simulink model "PX4_Receive"  (R2025b)
settings: Solver=FixedStepAuto  StartTime=0.0  StopTime=60  RelTol=1e-3
undefined symbols (not defined in the file or in its folder): acceleration, actuator, attitude, body_rate, codertarget, command, control, CustomLQR, FlightPlan, from_external, gcbh, HomeNED, HoverThrust, jerk, param1, param2, param3, pitch, pitch_body, position, PX4Params, PX4Tune, q_d, roll, roll_body, source_component, source_system, target_component, target_system, TestAmplitude, TestAxis, thrust_body, timestamp, timestamp_sample, TUNING_ON, TuningMaxClimbRate, TuningMinAltitude, TuningStage, TuningTestStart, velocity, yaw, yaw_body, yaw_sp_move_rate, yawspeed
libraries: px4Utilslib x53, px4uORBlib x52, simulink x13
(part 2 of 2)

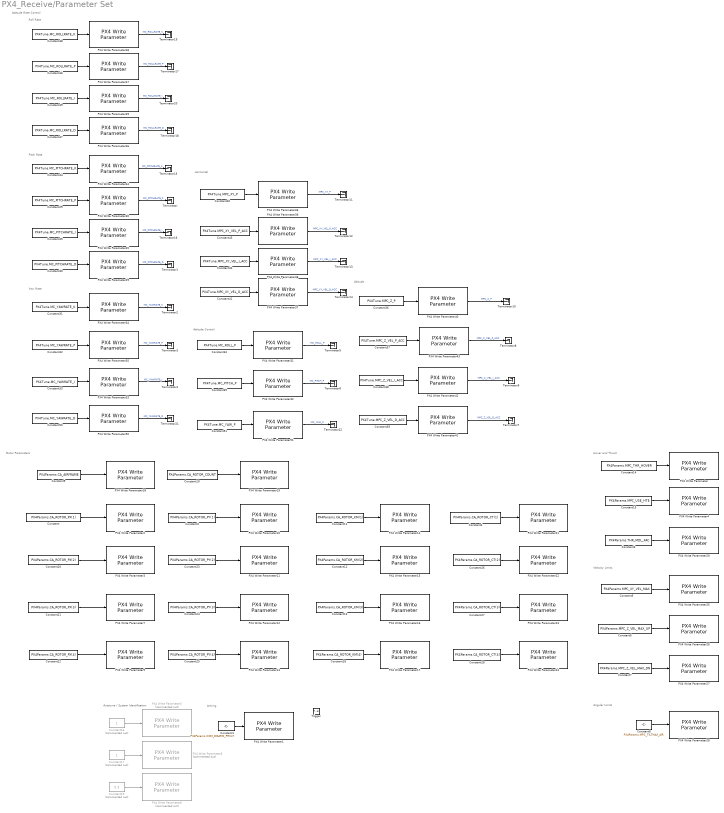
== system PX4_Receive/Parameter Set ==
  note: Yaw Rate
  note: Roll Rate
  note: Pitch Rate
  note: Horizontal
  note: Altitude
  note: Attitude Rate Control
  note: Arming
  note: Autotune / System Identification
  note: Hover and Thrust
  note: Motor Parameters
  note: Velocity Limits
  note: Angular Limits
  note: Attitude Control
  Trigger : TriggerPort  VariantControl=(inherit)  ShowOutputPort=on  PortDimensions=1
  Constant : Constant  Value=PX4Params.CA_ROTOR_PX(1)  OutDataTypeStr=single
  Constant1 : Constant  Value=PX4Params.COM_DISARM_PRFLT  OutDataTypeStr=single
  Constant10 : Constant  Value=PX4Params.CA_ROTOR_COUNT  OutDataTypeStr=int32
  Constant11 : Constant  Value=PX4Params.CA_ROTOR_KM(1)  OutDataTypeStr=single
  Constant12 : Constant  Value=PX4Params.CA_ROTOR_KM(2)  OutDataTypeStr=single
  Constant13 : Constant  Value=PX4Params.CA_ROTOR_KM(3)  OutDataTypeStr=single
  Constant14 : Constant  Value=PX4Params.MPC_THR_HOVER  OutDataTypeStr=single
  Constant15 : Constant  Value=PX4Params.MPC_USE_HTE  OutDataTypeStr=int32
  Constant16 : Constant  Commented=on  OutDataTypeStr=int32
  Constant17 : Constant  Commented=on  OutDataTypeStr=int32
  Constant18 : Constant  Value=PX4Params.CA_ROTOR_KM(4)  OutDataTypeStr=single
  Constant19 : Constant  Commented=on  Value=0.3  OutDataTypeStr=single
  Constant2 : Constant  Value=PX4Params.CA_ROTOR_PY(1)  OutDataTypeStr=single
  Constant20 : Constant  Value=PX4Params.CA_ROTOR_PX(2)  OutDataTypeStr=single
  Constant21 : Constant  Value=PX4Params.CA_ROTOR_PX(3)  OutDataTypeStr=single
  Constant22 : Constant  Value=PX4Params.CA_ROTOR_PX(4)  OutDataTypeStr=single
  Constant23 : Constant  Value=PX4Params.CA_ROTOR_PY(2)  OutDataTypeStr=single
  Constant24 : Constant  Value=PX4Params.CA_ROTOR_PY(3)  OutDataTypeStr=single
  Constant25 : Constant  Value=PX4Params.CA_ROTOR_PY(4)  OutDataTypeStr=single
  Constant26 : Constant  Value=PX4Params.CA_ROTOR_CT(2)  OutDataTypeStr=single
  Constant27 : Constant  Value=PX4Params.CA_ROTOR_CT(3)  OutDataTypeStr=single
  Constant28 : Constant  Value=PX4Params.CA_ROTOR_CT(4)  OutDataTypeStr=single
  Constant29 : Constant  Value=PX4Tune.MC_PITCHRATE_P  OutDataTypeStr=single
  Constant3 : Constant  Value=PX4Params.THR_MDL_FAC  OutDataTypeStr=single
  Constant30 : Constant  Value=PX4Tune.MC_PITCHRATE_D  OutDataTypeStr=single
  Constant31 : Constant  Value=PX4Tune.MC_YAWRATE_K  OutDataTypeStr=single
  Constant32 : Constant  Value=PX4Tune.MC_YAWRATE_P  OutDataTypeStr=single
  Constant33 : Constant  Value=PX4Tune.MC_YAWRATE_I  OutDataTypeStr=single
  Constant34 : Constant  Value=PX4Tune.MC_ROLL_P  OutDataTypeStr=single
  Constant35 : Constant  Value=PX4Tune.MC_PITCH_P  OutDataTypeStr=single
  Constant36 : Constant  Value=PX4Tune.MPC_Z_P  OutDataTypeStr=single
  Constant37 : Constant  Value=PX4Tune.MPC_Z_VEL_P_ACC  OutDataTypeStr=single
  Constant38 : Constant  Value=PX4Tune.MPC_Z_VEL_I_ACC  OutDataTypeStr=single
  Constant39 : Constant  Value=PX4Tune.MPC_Z_VEL_D_ACC  OutDataTypeStr=single
  Constant4 : Constant  Value=PX4Params.CA_ROTOR_CT(1)  OutDataTypeStr=single
  Constant40 : Constant  Value=PX4Tune.MPC_XY_P  OutDataTypeStr=single
  Constant41 : Constant  Value=PX4Tune.MPC_XY_VEL_D_ACC  OutDataTypeStr=single
  Constant42 : Constant  Value=PX4Tune.MPC_XY_VEL_I_ACC  OutDataTypeStr=single
  Constant43 : Constant  Value=PX4Tune.MPC_XY_VEL_P_ACC  OutDataTypeStr=single
  Constant44 : Constant  Value=PX4Tune.MC_PITCHRATE_K  OutDataTypeStr=single
  Constant45 : Constant  Value=PX4Tune.MC_PITCHRATE_I  OutDataTypeStr=single
  Constant46 : Constant  Value=PX4Tune.MC_ROLLRATE_P  OutDataTypeStr=single
  Constant47 : Constant  Value=PX4Tune.MC_ROLLRATE_D  OutDataTypeStr=single
  Constant48 : Constant  Value=PX4Tune.MC_ROLLRATE_K  OutDataTypeStr=single
  Constant49 : Constant  Value=PX4Tune.MC_ROLLRATE_I  OutDataTypeStr=single
  Constant5 : Constant  Value=PX4Params.MPC_XY_VEL_MAX  OutDataTypeStr=single
  Constant50 : Constant  Value=PX4Tune.MC_YAWRATE_D  OutDataTypeStr=single
  Constant51 : Constant  Value=PX4Tune.MC_YAW_P  OutDataTypeStr=single
  Constant6 : Constant  Value=PX4Params.MPC_Z_VEL_MAX_UP  OutDataTypeStr=single
  Constant7 : Constant  Value=PX4Params.MPC_Z_VEL_MAX_DN  OutDataTypeStr=single
  Constant8 : Constant  Value=PX4Params.MPC_TILTMAX_AIR  OutDataTypeStr=single
  Constant9 : Constant  Value=PX4Params.CA_AIRFRAME  OutDataTypeStr=int32
  PX4 Write Parameter : px4Utilslib/PX4 Write Parameter  ParameterName=MPC_THR_HOVER  outputStatus=off  SimulateUsing=Code generation
  PX4 Write Parameter1 : px4Utilslib/PX4 Write Parameter  ParameterName=COM_DISARM_PRFLT  outputStatus=off  SimulateUsing=Code generation
  PX4 Write Parameter10 : px4Utilslib/PX4 Write Parameter  ParameterName=CA_ROTOR0_PY  outputStatus=off  SimulateUsing=Code generation
  PX4 Write Parameter11 : px4Utilslib/PX4 Write Parameter  ParameterName=CA_ROTOR1_PY  outputStatus=off  SimulateUsing=Code generation
  PX4 Write Parameter12 : px4Utilslib/PX4 Write Parameter  ParameterName=CA_ROTOR2_PY  outputStatus=off  SimulateUsing=Code generation
  PX4 Write Parameter13 : px4Utilslib/PX4 Write Parameter  ParameterName=CA_ROTOR3_PY  outputStatus=off  SimulateUsing=Code generation
  PX4 Write Parameter14 : px4Utilslib/PX4 Write Parameter  ParameterName=CA_ROTOR0_KM  outputStatus=off  SimulateUsing=Code generation
  PX4 Write Parameter15 : px4Utilslib/PX4 Write Parameter  ParameterName=CA_ROTOR1_KM  outputStatus=off  SimulateUsing=Code generation
  PX4 Write Parameter16 : px4Utilslib/PX4 Write Parameter  ParameterName=CA_ROTOR2_KM  outputStatus=off  SimulateUsing=Code generation
  PX4 Write Parameter17 : px4Utilslib/PX4 Write Parameter  ParameterName=CA_ROTOR3_KM  outputStatus=off  SimulateUsing=Code generation
  PX4 Write Parameter18 : px4Utilslib/PX4 Write Parameter  ParameterName=CA_AIRFRAME  outputStatus=off  SimulateUsing=Code generation
  PX4 Write Parameter19 : px4Utilslib/PX4 Write Parameter  ParameterName=CA_ROTOR_COUNT  outputStatus=off  SimulateUsing=Code generation
  PX4 Write Parameter2 : px4Utilslib/PX4 Write Parameter  ParameterName=CA_ROTOR0_PX  outputStatus=off  SimulateUsing=Code generation
  PX4 Write Parameter20 : px4Utilslib/PX4 Write Parameter  ParameterName=THR_MDL_FAC  outputStatus=off  SimulateUsing=Code generation
  PX4 Write Parameter21 : px4Utilslib/PX4 Write Parameter  ParameterName=CA_ROTOR0_CT  outputStatus=off  SimulateUsing=Code generation
  PX4 Write Parameter22 : px4Utilslib/PX4 Write Parameter  ParameterName=CA_ROTOR1_CT  outputStatus=off  SimulateUsing=Code generation
  PX4 Write Parameter23 : px4Utilslib/PX4 Write Parameter  ParameterName=CA_ROTOR2_CT  outputStatus=off  SimulateUsing=Code generation
  PX4 Write Parameter24 : px4Utilslib/PX4 Write Parameter  ParameterName=CA_ROTOR3_CT  outputStatus=off  SimulateUsing=Code generation
  PX4 Write Parameter25 : px4Utilslib/PX4 Write Parameter  ParameterName=MPC_XY_VEL_MAX  outputStatus=off  SimulateUsing=Code generation
  PX4 Write Parameter26 : px4Utilslib/PX4 Write Parameter  ParameterName=MPC_Z_VEL_MAX_UP  outputStatus=off  SimulateUsing=Code generation
  PX4 Write Parameter27 : px4Utilslib/PX4 Write Parameter  ParameterName=MPC_Z_VEL_MAX_DN  outputStatus=off  SimulateUsing=Code generation
  PX4 Write Parameter28 : px4Utilslib/PX4 Write Parameter  ParameterName=MPC_TILTMAX_AIR  outputStatus=off  SimulateUsing=Code generation
  PX4 Write Parameter29 : px4Utilslib/PX4 Write Parameter  ParameterName=MC_PITCHRATE_D  outputStatus=on  SimulateUsing=Code generation
  PX4 Write Parameter3 : px4Utilslib/PX4 Write Parameter  ParameterName=CA_ROTOR1_PX  outputStatus=off  SimulateUsing=Code generation
  PX4 Write Parameter30 : px4Utilslib/PX4 Write Parameter  ParameterName=MC_PITCHRATE_P  outputStatus=on  SimulateUsing=Code generation
  PX4 Write Parameter31 : px4Utilslib/PX4 Write Parameter  ParameterName=MC_ROLL_P  outputStatus=on  SimulateUsing=Code generation
  PX4 Write Parameter32 : px4Utilslib/PX4 Write Parameter  ParameterName=MC_PITCH_P  outputStatus=on  SimulateUsing=Code generation
  PX4 Write Parameter33 : px4Utilslib/PX4 Write Parameter  ParameterName=MC_YAWRATE_I  outputStatus=on  SimulateUsing=Code generation
  PX4 Write Parameter34 : px4Utilslib/PX4 Write Parameter  ParameterName=MC_YAWRATE_K  outputStatus=on  SimulateUsing=Code generation
  PX4 Write Parameter35 : px4Utilslib/PX4 Write Parameter  ParameterName=MC_YAWRATE_P  outputStatus=on  SimulateUsing=Code generation
  PX4 Write Parameter36 : px4Utilslib/PX4 Write Parameter  ParameterName=MPC_XY_P  outputStatus=on  SimulateUsing=Code generation
  PX4 Write Parameter37 : px4Utilslib/PX4 Write Parameter  ParameterName=MPC_XY_VEL_D_ACC  outputStatus=on  SimulateUsing=Code generation
  PX4 Write Parameter38 : px4Utilslib/PX4 Write Parameter  ParameterName=MPC_XY_VEL_I_ACC  outputStatus=on  SimulateUsing=Code generation
  PX4 Write Parameter39 : px4Utilslib/PX4 Write Parameter  ParameterName=MPC_XY_VEL_P_ACC  outputStatus=on  SimulateUsing=Code generation
  PX4 Write Parameter4 : px4Utilslib/PX4 Write Parameter  ParameterName=MPC_USE_HTE  outputStatus=off  SimulateUsing=Code generation
  PX4 Write Parameter40 : px4Utilslib/PX4 Write Parameter  ParameterName=MPC_Z_P  outputStatus=on  SimulateUsing=Code generation
  PX4 Write Parameter41 : px4Utilslib/PX4 Write Parameter  ParameterName=MPC_Z_VEL_D_ACC  outputStatus=on  SimulateUsing=Code generation
  PX4 Write Parameter42 : px4Utilslib/PX4 Write Parameter  ParameterName=MPC_Z_VEL_I_ACC  outputStatus=on  SimulateUsing=Code generation
  PX4 Write Parameter43 : px4Utilslib/PX4 Write Parameter  ParameterName=MPC_Z_VEL_P_ACC  outputStatus=on  SimulateUsing=Code generation
  PX4 Write Parameter44 : px4Utilslib/PX4 Write Parameter  ParameterName=MC_PITCHRATE_K  outputStatus=on  SimulateUsing=Code generation
  PX4 Write Parameter45 : px4Utilslib/PX4 Write Parameter  ParameterName=MC_PITCHRATE_I  outputStatus=on  SimulateUsing=Code generation
  PX4 Write Parameter46 : px4Utilslib/PX4 Write Parameter  ParameterName=MC_ROLLRATE_D  outputStatus=on  SimulateUsing=Code generation
  PX4 Write Parameter47 : px4Utilslib/PX4 Write Parameter  ParameterName=MC_ROLLRATE_P  outputStatus=on  SimulateUsing=Code generation
  PX4 Write Parameter48 : px4Utilslib/PX4 Write Parameter  ParameterName=MC_ROLLRATE_K  outputStatus=on  SimulateUsing=Code generation
  PX4 Write Parameter49 : px4Utilslib/PX4 Write Parameter  ParameterName=MC_ROLLRATE_I  outputStatus=on  SimulateUsing=Code generation
  PX4 Write Parameter5 : px4Utilslib/PX4 Write Parameter  Commented=on  ParameterName=MC_AT_EN  outputStatus=off  SimulateUsing=Code generation
  PX4 Write Parameter50 : px4Utilslib/PX4 Write Parameter  ParameterName=MC_YAWRATE_D  outputStatus=on  SimulateUsing=Code generation
  PX4 Write Parameter51 : px4Utilslib/PX4 Write Parameter  ParameterName=MC_YAW_P  outputStatus=on  SimulateUsing=Code generation
  PX4 Write Parameter6 : px4Utilslib/PX4 Write Parameter  Commented=on  ParameterName=MC_AT_APPLY  outputStatus=off  SimulateUsing=Code generation
  PX4 Write Parameter7 : px4Utilslib/PX4 Write Parameter  ParameterName=CA_ROTOR2_PX  outputStatus=off  SimulateUsing=Code generation
  PX4 Write Parameter8 : px4Utilslib/PX4 Write Parameter  Commented=on  ParameterName=MC_AT_SYSID_AMP  outputStatus=off  SimulateUsing=Code generation
  PX4 Write Parameter9 : px4Utilslib/PX4 Write Parameter  ParameterName=CA_ROTOR3_PX  outputStatus=off  SimulateUsing=Code generation
  Terminator{,1..22} (23 alike) : Terminator
  wires:
  Constant19/1 -> PX4 Write Parameter8/1
  Constant17/1 -> PX4 Write Parameter6/1
  Constant14/1 -> PX4 Write Parameter/1
  Constant16/1 -> PX4 Write Parameter5/1
  Constant15/1 -> PX4 Write Parameter4/1
  Constant1/1 -> PX4 Write Parameter1/1
  Constant/1 -> PX4 Write Parameter2/1
  Constant21/1 -> PX4 Write Parameter7/1
  Constant2/1 -> PX4 Write Parameter10/1
  Constant22/1 -> PX4 Write Parameter9/1
  Constant9/1 -> PX4 Write Parameter18/1
  Constant11/1 -> PX4 Write Parameter14/1
  Constant12/1 -> PX4 Write Parameter15/1
  Constant13/1 -> PX4 Write Parameter16/1
  Constant18/1 -> PX4 Write Parameter17/1
  Constant10/1 -> PX4 Write Parameter19/1
  Constant3/1 -> PX4 Write Parameter20/1
  Constant5/1 -> PX4 Write Parameter25/1
  Constant6/1 -> PX4 Write Parameter26/1
  Constant7/1 -> PX4 Write Parameter27/1
  Constant8/1 -> PX4 Write Parameter28/1
  Constant20/1 -> PX4 Write Parameter3/1
  Constant23/1 -> PX4 Write Parameter11/1
  Constant24/1 -> PX4 Write Parameter12/1
  Constant25/1 -> PX4 Write Parameter13/1
  Constant4/1 -> PX4 Write Parameter21/1
  Constant26/1 -> PX4 Write Parameter22/1
  Constant27/1 -> PX4 Write Parameter23/1
  Constant28/1 -> PX4 Write Parameter24/1
  Constant29/1 -> PX4 Write Parameter30/1
  Constant30/1 -> PX4 Write Parameter29/1
  Constant31/1 -> PX4 Write Parameter34/1
  Constant32/1 -> PX4 Write Parameter35/1
  Constant33/1 -> PX4 Write Parameter33/1
  Constant35/1 -> PX4 Write Parameter32/1
  Constant34/1 -> PX4 Write Parameter31/1
  Constant36/1 -> PX4 Write Parameter40/1
  Constant39/1 -> PX4 Write Parameter41/1
  Constant38/1 -> PX4 Write Parameter42/1
  Constant37/1 -> PX4 Write Parameter43/1
  Constant40/1 -> PX4 Write Parameter36/1
  Constant41/1 -> PX4 Write Parameter37/1
  Constant42/1 -> PX4 Write Parameter38/1
  Constant43/1 -> PX4 Write Parameter39/1
  PX4 Write Parameter30/1 -> Terminator/1  "MC_PITCHRATE_P"
  PX4 Write Parameter29/1 -> Terminator1/1  "MC_PITCHRATE_D"
  PX4 Write Parameter35/1 -> Terminator3/1  "MC_YAWRATE_P"
  PX4 Write Parameter34/1 -> Terminator2/1  "MC_YAWRATE_K"
  PX4 Write Parameter33/1 -> Terminator4/1  "MC_YAWRATE_I"
  PX4 Write Parameter31/1 -> Terminator5/1  "MC_ROLL_P"
  PX4 Write Parameter32/1 -> Terminator6/1  "MC_PITCH_P"
  PX4 Write Parameter43/1 -> Terminator8/1  "MPC_Z_VEL_P_ACC"
  PX4 Write Parameter40/1 -> Terminator10/1  "MPC_Z_P"
  PX4 Write Parameter42/1 -> Terminator9/1  "MPC_Z_VEL_I_ACC"
  PX4 Write Parameter41/1 -> Terminator7/1  "MPC_Z_VEL_D_ACC"
  PX4 Write Parameter36/1 -> Terminator11/1  "MPC_XY_P"
  PX4 Write Parameter39/1 -> Terminator12/1  "MPC_XY_VEL_P_ACC"
  PX4 Write Parameter38/1 -> Terminator13/1  "MPC_XY_VEL_I_ACC"
  PX4 Write Parameter37/1 -> Terminator14/1  "MPC_XY_VEL_D_ACC"
  PX4 Write Parameter44/1 -> Terminator15/1  "MC_PITCHRATE_K"
  Constant44/1 -> PX4 Write Parameter44/1
  Constant45/1 -> PX4 Write Parameter45/1
  PX4 Write Parameter45/1 -> Terminator16/1  "MC_PITCHRATE_I"
  PX4 Write Parameter49/1 -> Terminator20/1  "MC_ROLLRATE_I"
  Constant48/1 -> PX4 Write Parameter48/1
  PX4 Write Parameter46/1 -> Terminator18/1  "MC_ROLLRATE_D"
  Constant47/1 -> PX4 Write Parameter46/1
  PX4 Write Parameter47/1 -> Terminator17/1  "MC_ROLLRATE_P"
  PX4 Write Parameter48/1 -> Terminator19/1  "MC_ROLLRATE_K"
  Constant46/1 -> PX4 Write Parameter47/1
  Constant49/1 -> PX4 Write Parameter49/1
  Constant50/1 -> PX4 Write Parameter50/1
  PX4 Write Parameter50/1 -> Terminator21/1  "MC_YAWRATE_D"
  Constant51/1 -> PX4 Write Parameter51/1
  PX4 Write Parameter51/1 -> Terminator22/1  "MC_YAW_P"

== system PX4_Receive/Custom Controller (LQR)/Disable land auto-disarm ==
  Trigger : TriggerPort  VariantControl=(inherit)  PortDimensions=1
  COM_DISARM_LAND : px4Utilslib/PX4 Write Parameter  ParameterName=COM_DISARM_LAND  outputStatus=off  SimulateUsing=Code generation
  Value : Constant  Value=single(-1)  OutDataTypeStr=single
  wires:
  Value/1 -> COM_DISARM_LAND/1

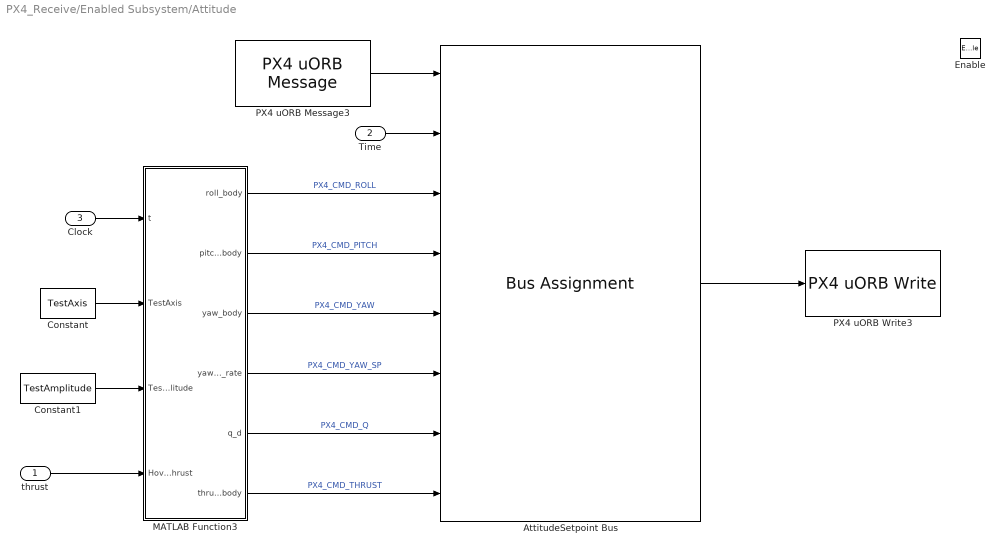
== system PX4_Receive/Enabled Subsystem/Attitude ==
  thrust : Inport
  Time : Inport  Port=2
  Clock : Inport  Port=3
  Enable : EnablePort
  AttitudeSetpoint Bus : BusAssignment  AssignedSignals=timestamp,roll_body,pitch_body,yaw_body,yaw_sp_move_rate,q_d,thrust_body
  Constant : Constant  Value=TestAxis
  Constant1 : Constant  Value=TestAmplitude
  MATLAB Function3 : MATLAB Function  TreatAsAtomicUnit=on
  PX4 uORB Message3 : px4uORBlib/PX4 uORB Message  uORBTopic=VehicleAttitudeSetpoint  SampleTime=-1  selectInstance=vehicle_attitude_setpoint
  PX4 uORB Write3 : px4uORBlib/PX4 uORB Write  uORBTopic=VehicleAttitudeSetpoint  selectInstance=vehicle_attitude_setpoint  MessageQueueLen=1
  wires:
  MATLAB Function3/5(q_d) -> AttitudeSetpoint Bus/7  "PX4_CMD_Q"
  Constant/1 -> MATLAB Function3/2(TestAxis)
  MATLAB Function3/1(roll_body) -> AttitudeSetpoint Bus/3  "PX4_CMD_ROLL"
  PX4 uORB Message3/1 -> AttitudeSetpoint Bus/1
  MATLAB Function3/2(pitch_body) -> AttitudeSetpoint Bus/4  "PX4_CMD_PITCH"
  MATLAB Function3/4(yaw_sp_move_rate) -> AttitudeSetpoint Bus/6  "PX4_CMD_YAW_SP"
  MATLAB Function3/3(yaw_body) -> AttitudeSetpoint Bus/5  "PX4_CMD_YAW"
  Time/1 -> AttitudeSetpoint Bus/2
  AttitudeSetpoint Bus/1 -> PX4 uORB Write3/1
  Constant1/1 -> MATLAB Function3/3(TestAmplitude)
  MATLAB Function3/6(thrust_body) -> AttitudeSetpoint Bus/8  "PX4_CMD_THRUST"
  thrust/1 -> MATLAB Function3/4(HoverThrust)
  Clock/1 -> MATLAB Function3/1(t)

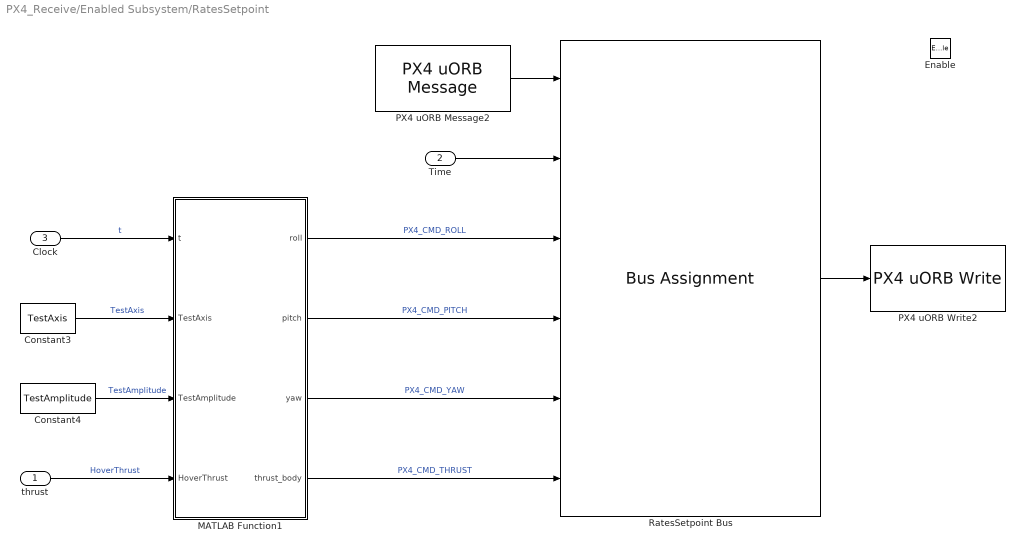
== system PX4_Receive/Enabled Subsystem/RatesSetpoint ==
  thrust : Inport
  Time : Inport  Port=2
  Clock : Inport  Port=3
  Enable : EnablePort
  Constant3 : Constant  Value=TestAxis
  Constant4 : Constant  Value=TestAmplitude
  MATLAB Function1 : MATLAB Function  TreatAsAtomicUnit=on
  PX4 uORB Message2 : px4uORBlib/PX4 uORB Message  uORBTopic=VehicleRatesSetpoint  SampleTime=-1  selectInstance=VehicleRatesSetpoint
  PX4 uORB Write2 : px4uORBlib/PX4 uORB Write  uORBTopic=VehicleRatesSetpoint  selectInstance=VehicleRatesSetpoint  MessageQueueLen=1
  RatesSetpoint Bus : BusAssignment  AssignedSignals=timestamp,roll,pitch,yaw,thrust_body
  wires:
  Time/1 -> RatesSetpoint Bus/2
  thrust/1 -> MATLAB Function1/4(HoverThrust)  "HoverThrust"
  MATLAB Function1/4(thrust_body) -> RatesSetpoint Bus/6  "PX4_CMD_THRUST"
  MATLAB Function1/1(roll) -> RatesSetpoint Bus/3  "PX4_CMD_ROLL"
  Constant4/1 -> MATLAB Function1/3(TestAmplitude)  "TestAmplitude"
  Constant3/1 -> MATLAB Function1/2(TestAxis)  "TestAxis"
  PX4 uORB Message2/1 -> RatesSetpoint Bus/1
  MATLAB Function1/3(yaw) -> RatesSetpoint Bus/5  "PX4_CMD_YAW"
  MATLAB Function1/2(pitch) -> RatesSetpoint Bus/4  "PX4_CMD_PITCH"
  RatesSetpoint Bus/1 -> PX4 uORB Write2/1
  Clock/1 -> MATLAB Function1/1(t)  "t"

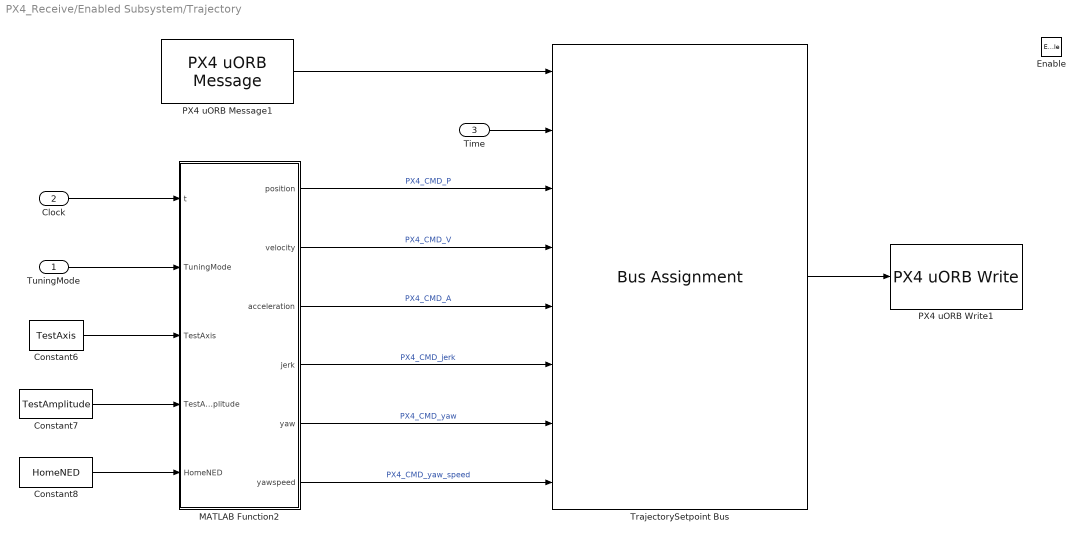
== system PX4_Receive/Enabled Subsystem/Trajectory ==
  TuningMode : Inport
  Clock : Inport  Port=2
  Time : Inport  Port=3
  Enable : EnablePort
  Constant6 : Constant  Value=TestAxis
  Constant7 : Constant  Value=TestAmplitude
  Constant8 : Constant  Value=HomeNED
  MATLAB Function2 : MATLAB Function  TreatAsAtomicUnit=on
  PX4 uORB Message1 : px4uORBlib/PX4 uORB Message  uORBTopic=TrajectorySetpoint  SampleTime=-1  selectInstance=TrajectorySetpoint
  PX4 uORB Write1 : px4uORBlib/PX4 uORB Write  uORBTopic=TrajectorySetpoint  selectInstance=TrajectorySetpoint  MessageQueueLen=1
  TrajectorySetpoint Bus : BusAssignment  AssignedSignals=timestamp,position,velocity,acceleration,jerk,yaw,yawspeed
  wires:
  MATLAB Function2/2(velocity) -> TrajectorySetpoint Bus/4  "PX4_CMD_V"
  Time/1 -> TrajectorySetpoint Bus/2
  Constant8/1 -> MATLAB Function2/5(HomeNED)
  Constant7/1 -> MATLAB Function2/4(TestAmplitude)
  MATLAB Function2/5(yaw) -> TrajectorySetpoint Bus/7  "PX4_CMD_yaw"
  TuningMode/1 -> MATLAB Function2/2(TuningMode)
  MATLAB Function2/6(yawspeed) -> TrajectorySetpoint Bus/8  "PX4_CMD_yaw_speed"
  MATLAB Function2/1(position) -> TrajectorySetpoint Bus/3  "PX4_CMD_P"
  MATLAB Function2/4(jerk) -> TrajectorySetpoint Bus/6  "PX4_CMD_jerk"
  TrajectorySetpoint Bus/1 -> PX4 uORB Write1/1
  PX4 uORB Message1/1 -> TrajectorySetpoint Bus/1
  MATLAB Function2/3(acceleration) -> TrajectorySetpoint Bus/5  "PX4_CMD_A"
  Constant6/1 -> MATLAB Function2/3(TestAxis)
  Clock/1 -> MATLAB Function2/1(t)

== matlab function PX4_Receive/Enabled Subsystem/Attitude/MATLAB Function3 ==
  data: roll_body output; t input; pitch_body output; TestAxis input; TestAmplitude input; HoverThrust input; yaw_body output; yaw_sp_move_rate output; q_d output; thrust_body output

function [roll_body, pitch_body, yaw_body, ...
          yaw_sp_move_rate, q_d, thrust_body] = ...
    attitude_test(t, TestAxis, TestAmplitude, HoverThrust)
%#codegen
% Automated attitude controller tests.
%
% Inputs:
% t             - Elapsed test time [s]
% TestAxis      - 1=Roll, 2=Pitch, 3=Yaw
% TestAmplitude - Attitude amplitude [rad]
% HoverThrust   - Normalized hover thrust magnitude [0,1]

roll_body  = single(0);
pitch_body = single(0);
yaw_body   = single(0);

yaw_sp_move_rate = single(0);

% Positive and negative attitude steps
[axisNow,segmentTime,segmentAmplitude]=px4_tuning_segment(t,uint8(2),TestAxis,TestAmplitude);
cmd=px4_tuning_step_command(segmentTime,uint8(2),segmentAmplitude);

switch axisNow
    case 1
        roll_body = cmd;
    case 2
        pitch_body = cmd;
    case 3
        yaw_body = cmd;
end

% Euler ZYX -> quaternion
% PX4 uses scalar-first ordering [w; x; y; z]

cr = cos(double(roll_body)/2);
sr = sin(double(roll_body)/2);

cp = cos(double(pitch_body)/2);
sp = sin(double(pitch_body)/2);

cy = cos(double(yaw_body)/2);
sy = sin(double(yaw_body)/2);


% Quaternion [w, x, y, z] - row vector [1x4]
q_d = single([
    cr*cp*cy + sr*sp*sy, ...
    sr*cp*cy - cr*sp*sy, ...
    cr*sp*cy + sr*cp*sy, ...
    cr*cp*sy - sr*sp*cy
]);


% Normalized thrust command
thrust = min(max(single(HoverThrust), single(0)), single(1));
thrust_body = single([0; 0; -double(thrust)]');
end

== matlab function PX4_Receive/Custom Controller (LQR)/LQR ==
  data: t input; control output; pos input; vel input; q input; omega input; mcmd output; xerr output; FlightPlan parameter; CustomLQR parameter
function [control,mcmd,xerr] = fcn(t,pos,vel,q,omega,FlightPlan, CustomLQR)
%#codegen
% 12-state hover LQR (custom controller). See lqr_hover_control.m and custom_controller_parameters.m.
[control,mcmd,xerr] = lqr_hover_control(t,pos,vel,q,omega,FlightPlan,CustomLQR);
end

== matlab function PX4_Receive/Enabled Subsystem/MATLAB Function2 ==
  data: z_ned input; thrust output; vz_ned input; HoverThrust input; HomeNED parameter

function thrust = test_altitude_thrust(z_ned, vz_ned, HoverThrust, HomeNED)
%#codegen
%
% Independent altitude-hold test harness.
% Used during rate and attitude tuning.
%
% Inputs:
% z_ned       = Estimated local position Z [m]
% vz_ned      = Estimated vertical velocity [m/s]
% HoverThrust = Normalized hover thrust (from SimParams.HoverThrustFraction)
%
% Output:
% thrust      = Normalized collective thrust [0,1]
%
% NED conventions:
% z < 0 corresponds to altitude above the origin.
% vz < 0 corresponds to upward motion.

%% Settings

h_ref = -double(HomeNED(3));       % Desired altitude [m]

Kp = 0.8;           % [1/s^2]
Kd = 1.6;           % [1/s]

g = 9.82;

a_max = 4.0;        % Maximum desired acceleration [m/s^2]

%% Convert NED to altitude convention

h = -double(z_ned);
vh = -double(vz_ned);

%% Altitude PD

e = h_ref - h;

a_cmd = Kp*e - Kd*vh;

%% Limit desired acceleration

a_cmd = min(max(a_cmd,-a_max),a_max);

%% Convert desired acceleration to collective thrust

thrust = double(HoverThrust)*(1.0 + a_cmd/g);

%% Saturation

thrust = min(max(thrust,0.10),0.55);

end

== matlab function PX4_Receive/Enabled Subsystem/MATLAB Function1 ==
  data: t input; TuningMode output; TestTime output; TuningStage input; z input; vz input; TuningTestStart parameter; FlightPlan parameter; TuningMinAltitude parameter; TuningMaxClimbRate parameter
function [TuningMode,TestTime]=tuning_schedule(t,TuningStage,z,vz,TuningTestStart,FlightPlan,TuningMinAltitude,TuningMaxClimbRate)
%#codegen
persistent clockOrigin
if isempty(clockOrigin),clockOrigin=double(t)*1e-6;end
elapsed=double(t)*1e-6-clockOrigin;
[TuningMode,TestTime]=px4_tuning_schedule(elapsed,TuningStage,TuningTestStart,z,vz,FlightPlan,TuningMinAltitude,TuningMaxClimbRate);
end

== matlab function PX4_Receive/MATLAB Function2 ==
  data: t input; position output; velocity output; acceleration output; jerk output; yaw output; yawspeed output; FlightPlan parameter
function [position,velocity,acceleration,jerk,yaw,yawspeed] = fcn(t, FlightPlan)
%#codegen
[position,velocity,acceleration,jerk,yaw,yawspeed] = flight_trajectory(t,FlightPlan);
end

== matlab function PX4_Receive/Enabled Subsystem/Trajectory/MATLAB Function2 ==
  data: t input; position output; velocity output; acceleration output; jerk output; yaw output; yawspeed output; TuningMode input; TestAxis input; TestAmplitude input; HomeNED input; FlightPlan parameter; TuningTestStart parameter
function [position,velocity,acceleration,jerk,yaw,yawspeed]=trajectory_test(t,TuningMode,TestAxis,TestAmplitude,HomeNED,FlightPlan,TuningTestStart)
%#codegen
[position,velocity,acceleration,jerk,yaw,yawspeed]=px4_tuning_trajectory(t,TuningMode,TestAxis,TestAmplitude,HomeNED,FlightPlan,TuningTestStart);
end

== matlab function PX4_Receive/Enabled Subsystem/MATLAB Function ==
  data: TuningMode input; position output; velocity output; acceleration output; attitude output; body_rate output; actuator output

function [position, velocity, acceleration, attitude, body_rate, actuator] = offboard_control_mode(TuningMode)
%#codegen
% OFFBOARD_CONTROL_MODE
% Selects the PX4 Offboard control mode for automated tuning.
%
% TuningMode:
%   0 = Disabled
%   1 = Angular-rate tuning (roll, pitch, yaw)
%   2 = Attitude tuning (roll, pitch, yaw)
%   3 = Velocity tuning (XY and Z)
%   4 = Position tuning (XY and Z)
%   5 = Acceleration control
%   6 = Direct actuator control

% Initialize all modes as disabled
position     = false;
velocity     = false;
acceleration = false;
attitude     = false;
body_rate    = false;
actuator     = false;

switch TuningMode

    case 1
        % Angular-rate PID tuning
        body_rate = true;

    case 2
        % Attitude controller tuning
        attitude = true;

    case 3
        % Velocity controller tuning
        velocity = true;

    case 4
        % Position controller tuning
        position = true;

    case 5
        % Acceleration control
        acceleration = true;

    case 6
        % Direct actuator control
        actuator = true;

    otherwise
        % Disabled: all fields remain false
end

end

== matlab function PX4_Receive/Enabled Subsystem/RatesSetpoint/MATLAB Function1 ==
  data: t input; roll output; TestAxis input; TestAmplitude input; HoverThrust input; pitch output; yaw output; thrust_body output

function [roll, pitch, yaw, thrust_body] = ...
    rate_test(t, TestAxis, TestAmplitude, HoverThrust)
%#codegen
%
% TestAxis:
%   1 = Roll rate
%   2 = Pitch rate
%   3 = Yaw rate
%
% t = TestTime from tuning_schedule
%
% Outputs are SINGLE to match PX4 uORB bus fields.

%% Initialize outputs

roll  = single(0);
pitch = single(0);
yaw   = single(0);

%% Test amplitude

A = single(TestAmplitude);
r = single(0);

%% Rate excitation
[axisNow,segmentTime,segmentAmplitude]=px4_tuning_segment(t,uint8(1),TestAxis,TestAmplitude);
r=px4_tuning_step_command(segmentTime,uint8(1),segmentAmplitude);

%% Select axis

if axisNow == 1

    roll = r;

elseif axisNow == 2

    pitch = r;

elseif axisNow == 3

    yaw = r;

end

%% Collective thrust

thrust = single(HoverThrust);
thrust = min(max(thrust,single(0)),single(1));

thrust_body = single([0; 0; -thrust]');

end
